simulink model "DC_motor"  (R2025b)
settings: Solver=VariableStepAuto  StartTime=0.0  StopTime=10.0  RelTol=1e-3
values from neighbouring files (symbols this model uses):
  b = 0.00224986588705    [motorbike_chars.mat]    (also in motorbike_cruise_control.mat)
  J = 9.9e-07    [loads.mat]    (also in loads_new_cell.mat; motorbike_chars.mat = 0.000153; motorbike_cruise_control.mat = 0.000153)
  K_e = 0.0065    [loads.mat]    (also in loads_new_cell.mat; motorbike_chars.mat = 0.12; motorbike_cruise_control.mat = 0.12)
  L_a = 0.002    [loads.mat]    (also in loads_new_cell.mat; motorbike_chars.mat = 0.00265; motorbike_cruise_control.mat = 0.00265)
  R_a = 6.5    [loads.mat]    (also in loads_new_cell.mat; motorbike_chars.mat = 13.1; motorbike_cruise_control.mat = 13.1)
settings Model: Creator=konstantinos  LastModifiedBy=konstantinos

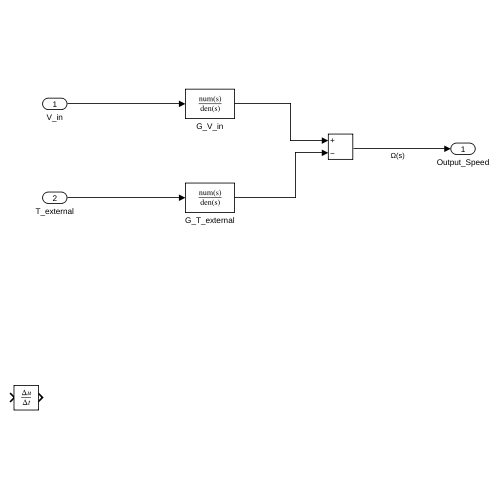
[thumbnail: Simulink's stored preview of the top-level diagram]
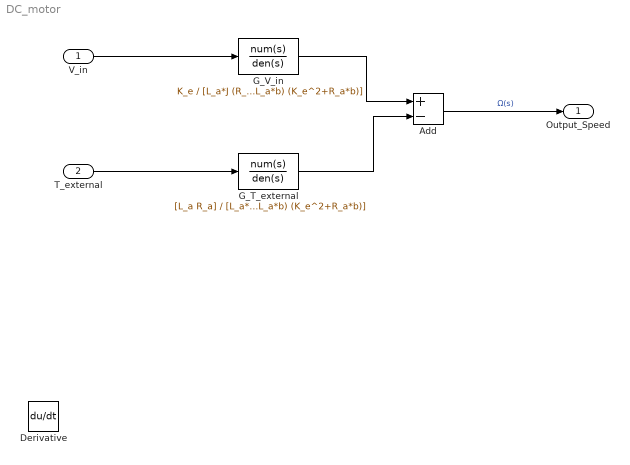
== system DC_motor ==
  V_in : Inport
  T_external : Inport  Port=2
  Add : Sum  Inputs=+-
  Derivative : Derivative
  G_T_external : TransferFcn  Numerator=[L_a R_a]  Denominator=[L_a*J (R_a*J+L_a*b) (K_e^2+R_a*b)]
  G_V_in : TransferFcn  Numerator=K_e  Denominator=[L_a*J (R_a*J+L_a*b) (K_e^2+R_a*b)]
  Output_Speed : Outport
  wires:
  Add/1 -> Output_Speed/1  "Ω(s)"
  V_in/1 -> G_V_in/1
  T_external/1 -> G_T_external/1
  G_V_in/1 -> Add/1
  G_T_external/1 -> Add/2
